simulink model "BimanualCarvingModified"  (R2013a)
settings: Solver=ode4  SolverMode=SingleTasking  StartTime=0.0  StopTime=inf  FixedStep=0.0005  RelTol=1e-3
StartFcn:
  |  warndlg('Dexterit-E models cannot run under simulation. Please compile your model and run it from within Dexterit-E.');set_param(bdroot,'SimulationCommand','stop')
model workspace (MAT data in the model file):
  BKIN_STEP_TIME = 0.0005
  col_x = 1
  col_y = 2
  WIDTH = 3
  HEIGHT = 4
  TARGET_COL = 1
  LOAD = 2
  TRAJ_DURATION_COL = 3
  MAX_LOAD = 2
  FORCE_ON = 1
  HAND_RADIUS = 6
  REST_COL = 4
  TRAINING_COL = 5
  HAND_COLOR = 5
  TARGET_STROKE = 8
  TARGET_RADIUS = 9
  xMaxCursor = 15
  yMaxCursor = 16
  TARGET_COLOR = 7
  START_X = 10
  START_Y = 11
  STIFFNESS_MATERIAL = 3
  MATERIAL_MASS = 4
  MATERIAL_DAMPING = 5
  STIFFNESS_HANDS = 6
  MATERIAL_GOAL_COLOR = 12
  SCALE_VIBRATION = 7
  STONE_WIDTH = 6
  MATERIAL_DUCTILITY = 8
  TARG_COLOR = 1
  TEXT_COLOR = 13
  TEXTBOX_WIDTH = 14
  TEXTBOX_HEIGHT = 15
  ROTATION = 16
  LABEL_TEXT = 17
  LABEL_COLOR = 18
  LABEL_HEIGHT = 19
  ADVANCE_EMG_PLACEMENT = 2
  ADVANCE_EMG_MAX = 3
  EMG_ADVANCE_BUTTON = 1
  EMG_MVC_BUTTON = 2
  START_TRIAL = 3
  END_TRIAL = 4
  MUSC_NUM = 2
  HAND_DISTANCE = 3
  SYN_NUM = 4
  IS_R2_REAL = 5
  R2_SCORE_SD = 6
undefined symbols (not defined in the file or in its folder): slselsubs
libraries: xpclib x9, simulink x6, General x3, KINARM_loads x2, Video x2, KINARM_IO x1, KINARM_EP_loads x1
(part 4 of 6)

== matlab function BimanualCarvingModified/Draw_target/MATLAB Function ==
  data: target input; VCODE output; state_in input; target_type input; opacity_in input; target_display input; x_index input; y_index input; num_states input; stateindices input; target_labels input; KINData input; yWall input; trial_state input; stoneWidth input
function VCODE = fcn(target, state_in, target_type, opacity_in, target_display, x_index, y_index, num_states, stateindices, target_labels, KINData, yWall, trial_state,stoneWidth)

% stateindices should follow this order (depending on target-type):
% 1: fill colour
% 2: stroke colour
% 3: stroke width
% 4: major radius / radius / start point (line)
% 5: minor radius / end point (line)
% 6: orientation angle



% VCODEs are length 70. All units in a VCODE should be SI, e.g. (m) and (rad). Elements in a VCODE are defined as follows:
%
% For all target types:
%  1: target type
%       1 - circle
%       2 - ellipse
%       3 - rectangle
%       4 - line
%       5 - triangle
%       11 - circle with label
%       12 - ellipse with label
%       13 - rectangle with label
%       14 - line with label
%       15 - triangle with label
%  2: target on/off status and target display (which display target will appear on)
%		0 - off
%		1 - on, appearing on both subject and operator displays
%       2 - on, appearing on subject display only
%       3 - on, appearing on operator display only
%  3: x position (m)
%  4: y position (m)
%  5: fill colour (RRGGBB) or texture index
%  6: stroke colour (RRGGBB) or texture index
%  7: stroke width
%  8: reserved for target background ID
%  9: opacity
%
% For circles:
%  10: radius (m)
%
% For ellipses:
%  10: major radius (m)
%  11: minor radius (m)
%  12: orientation of major axis (rad)
%
% For rectangles:
%  10: length (m)
%  11: height (m)
%  12: orientation (rad) (relative to x, y already shown)
%
% For lines:
%  10: endpoint x-axis coordinate relative to start point (m)
%  11: endpoint y-axis coordinate relative to start point (m)
%
% For triangles:
%  10: length (m)
%  11: height (m)
%  12: offset of peak from midpoint of length (m)
%  13: orientation (rad)
%
% For all labelled target types:
%  14: reserved
%  15-64: label characters (indexes in ISO 8859-1 character set)
%  65: label colour (0xRRGGBB), opacity is set by the vcode's opacity (9).
%  66: label height (m)
%  67: reserved
%  68: reserved
%  69: reserved
%  70: reserved

num_targets = 4;
stoneLength = 0.1;

% NOTE: we assume that the STATE and/or OPACITY inputs are vectors. 

% If the length of the input STATE is not the same as the number of targets then make STATE a column vector of the same length as 
% the TARGET input, using the first STATE (i.e. all targets get the same state)
if num_targets == length(state_in)
	state = reshape(state_in, num_targets, 1);
else
	state = state_in(1) * ones(num_targets, 1);
end


% If the length of the input OPACITY is not the same as the number of targets then make OPACITY a column vector of the same length as
% the TARGET input, using the first OPACITY (i.e. all targets get the same opacity)
if num_targets == length(opacity_in)
	opacity = reshape(opacity_in, num_targets, 1);
else
	opacity = opacity_in(1) * ones(num_targets, 1);
end


% Clamping the opacity to [0, 100].
opacity = min(opacity, 100);
opacity = max(opacity, 0);

VCODE = zeros(num_targets, 70);

% Set the target type. Targets with labels have type codes 10 greater than their unlabelled counterparts.
VCODE(:, 1) = target_type + 10;
VCODE(:, 2) = target_display;

VCODE(:, 5) = colourshift(target(1, stateindices(state(1), 1)));
VCODE(:, 6) = colourshift(target(1, stateindices(state(1), 1)));

% Set the opacity value
VCODE(:, 9) = opacity_in(1);
% Target only visible during tracking in trial_state==2
if trial_state==0
    VCODE(:, 5) = colourshift(1000000000);
    VCODE(:, 6) = colourshift(1000000000);
    VCODE(:, 9) = 0;
end


% Stroke width
VCODE(:, 7) = target(1, stateindices(state(1), 3))*0.01 * 2;

VCODE(:, 3) = [-stoneWidth/2;stoneWidth/2;stoneWidth/2;-stoneWidth/2];  % x position (m)
VCODE(:, 4) = [yWall;yWall;yWall+stoneLength;yWall+stoneLength];  % y position (m)

VCODE(:, 10) = [stoneWidth;0;-stoneWidth;0];  % line endpoint in x axis, relative to start (m)
VCODE(:, 11) = [0;stoneLength;0;-stoneLength];  % line endpoint in y axis, relative to start (m)

%{
persistent TargetIndex;
if isempty(TargetIndex), TargetIndex = 1; end
% Set the hand position.
if TargetIndex<=length(xMaterial)
    % Initially draw the whole material from left to right
    % Line beginning
    VCODE(:, 3) = xMaterial(TargetIndex);  % x position (m)
    VCODE(:, 4) = yMaterial(TargetIndex);  % y position (m)
    
    % Line endpoint
    VCODE(:, 10) = xMaterial(TargetIndex+1)-VCODE(:,3);  % line endpoint in x axis, relative to start (m)
    VCODE(:, 11) = yMaterial(TargetIndex+1)-VCODE(:,4);  % line endpoint in y axis, relative to start (m)
else
    % After material is all drawn, update only the changing section
    % Line beginning
    VCODE(:, 3) = xMaterial(MaterialUpdateInd1);  % x position (m)
    VCODE(:, 4) = yMaterial(MaterialUpdateInd1);  % y position (m)
    
    % Line endpoint
    VCODE(:, 10) = xMaterial(MaterialUpdateInd2)-VCODE(:,3);  % line endpoint in x axis, relative to start (m)
    VCODE(:, 11) = yMaterial(MaterialUpdateInd2)-VCODE(:,4);  % line endpoint in y axis, relative to start (m)
end


TargetIndex = min(length(xMaterial)+5,TargetIndex+1);
%}
%{
for ii = 1:num_targets
	% Set the target on/off state. If the state input is 0, the target is off. Users of the VCODE should respect this
	% as an indication that the rest of the VCODE will be uninitialized.
	if (state(ii) <= 0) || (state(ii) > num_states)
		VCODE(ii, 2) = 0;  % target is off
	else
		VCODE(ii, 2) = target_display;  % Default is that target is on; target displays as specified by block mask
	end

	fill_colour_col = stateindices(state(ii), 1);
	stroke_colour_col = stateindices(state(ii), 2);
	stroke_width_col = stateindices(state(ii), 3);
	
	% Set the fill colour. Fill colour currently comes from the GUI in RRRGGGBBB format.
	%{
    if fill_colour_col == 0
		VCODE(ii, 5) = -2^31;
	elseif target(fill_colour_col) < 0
		VCODE(ii, 5) = target(ii, fill_colour_col);
	else
		VCODE(ii, 5) = colourshift(target(ii, fill_colour_col));
    end
    %}
    VCODE(ii,5) = colourshift(1000000000);
	
	% Set the stroke colour. Stroke colour currently comes from the GUI in RRRGGGBBB format.
    if trial_state==1
        if stroke_colour_col == 0
            VCODE(ii, 6) = -2^31;
        elseif target(stroke_colour_col) < 0
            VCODE(ii, 6) = target(ii, stroke_colour_col);
        else
            VCODE(ii, 6) = colourshift( target(ii, stroke_colour_col) );
        end
    else
        % CIRCLE APPEARS ONLY DURING TASK
        VCODE(ii, 6) = colourshift(1000000000);
    end

	% Set the stroke width. if target table index for stroke width is zero, then the stroke width is undefined
	if stroke_width_col == 0
		VCODE(ii, 7) = 0;                   % if stroke width column is 0, then stroke width is 0
	elseif stroke_width_col < 0
		VCODE(ii, 7) = 0.001;               % if stroke width column is -ve, then a 1mm default is chosen
	else
		VCODE(ii, 7) = target(ii, stroke_width_col) * 0.01;  % if stroke width column is +ve, convert width from (cm) in target table to (m)
    end

	% Set the opacity value
	VCODE(ii, 9) = opacity(ii);

	% Set attributes specific to each target type. In the process, note the first state vector column used for label information.
	label_index = 1;

	% Set attributes specific to each target type.
	if target_type == 1

		% Handle circle target:
		radius_col = stateindices(state(ii), 4);
		VCODE(ii, 10)=target(ii, radius_col);  % radius (in m)
	    label_index = 5;

	elseif target_type == 2 || target_type == 3

	    % Handle ellipse or rectangle target:
		major_col = stateindices(state(ii), 4);
		minor_col = stateindices(state(ii), 5);
		orientation_col = stateindices(state(ii), 6);
		
		VCODE(ii, 10) = target(ii, major_col) * 0.01;  % major radius (convert from (cm) in target table to (m))
		VCODE(ii, 11) = target(ii, minor_col) * 0.01;  % minor radius (convert from (cm) in target table to (m))
		if orientation_col == 0
			VCODE(ii, 12) = 0;  % if orientation column is 0, set orientation to 0 rad
		else
			VCODE(ii, 12) = mod(target(ii, orientation_col), 360) * pi / 180.0;  % orientation (convert from (degrees) in target table to (rad))
		end
	    label_index = 7;
	
	elseif target_type == 4

		% Handle line target:
		%xendpoint_col = stateindices(state(ii), 4);
		%yendpoint_col = stateindices(state(ii), 5);
		VCODE(ii, 10) = 0;  % line endpoint in x axis, relative to start (m)
		VCODE(ii, 11) = stateindices(state(ii), 1);  % line endpoint in y axis, relative to start (taken from Target Table)
	    label_index = 6;

	elseif target_type == 5

		% Handle triangle target:
		length_col = stateindices(state(ii), 4);
		height_col = stateindices(state(ii), 5);
		offset_col = stateindices(state(ii), 6);
		orientation_col = stateindices(state(ii), 7);

		VCODE(ii, 10) = target(ii, length_col) * 0.01;  % length (convert from (cm) in target table to (m))

		% If the height column is set to 0 then the triangle is automatically made equilateral, with the base length used as length
		% for all sides. If the height column is non-zero, separate values for height and peak offset are taken from the target table.
		if height_col == 0
			VCODE(ii, 11) = sin(pi / 3.0) * VCODE(ii, 10);  % height for equilateral triangle
			VCODE(ii, 12) = 0;                          % peak offset for equilateral triangle
		else
			VCODE(ii, 11) = target(ii, height_col) * 0.01;  % height (convert from (cm) in target table to (m))
			VCODE(ii, 12) = target(ii, offset_col) * 0.01;  % peak offset (convert from (cm) in target table to (m))
		end

		if orientation_col == 0
			VCODE(ii, 13) = 0;  % if orientation column is 0, set orientation to 0 rad
		else
			VCODE(ii, 13) = mod(target(ii, orientation_col), 360) * pi / 180.0;  % orientation (convert from (degrees) in target table to (rad))
		end
	    label_index = 8;
		
	end
	
	% Copy the label characters to the VCODE.
	for jj = 1:50
		VCODE(ii, jj + 14) = target_labels( target( ii, stateindices(state(ii), label_index) ), jj );
	end

	% Set the label colour. Like other colours, label colour comes from the GUI in RRRGGGBBB format and is converted to a 32-bit
	% 0xRRGGBB value here. If the target column table index for the colour is 0, the label is transparent.
	if stateindices(state(ii), label_index + 1) == 0
		VCODE(ii, 65) = -2^31;
	elseif target( ii, stateindices(state(ii), label_index + 1) ) < 0
		VCODE(ii, 65) = target( ii, stateindices(state(ii), label_index + 1) );
	else
		VCODE(ii, 65) = colourshift( target( ii, stateindices(state(ii), label_index + 1) ) );
	end

	% Set the label height. Label height is converted from (cm) in the target table to (m).
	VCODE(ii, 66) = target( ii, stateindices(state, label_index + 2) ) * 0.01;


	
end
%}
% The colourshift function converts an "RRRGGGBBB" colour value to RRGBB (as an uint32).
function RRGGBBAA = colourshift(RRRGGGBBB)

%this is "no fill"
if RRRGGGBBB == 1000000000
    RRGGBBAA = cast(16777216, 'uint32'); %hex 0x1000000
    return; 
end

blue = cast(mod(RRRGGGBBB, 1000), 'uint32');
green = cast(mod(RRRGGGBBB - blue, 1000000) / 1000, 'uint32');
red = cast((RRRGGGBBB - (green * 1000) - blue) / 1000000, 'uint32');

RRGGBBAA = bitshift(red, 16) + bitshift(green, 8) + blue;

== matlab function BimanualCarvingModified/Trajectory subsystem/Create_Trajectory/Virtual_Trajectory/Extract_Position ==
  settings: fimath=|
      | fimath(...
      | 'RoundMode', 'floor',...
      | 'OverflowMode', 'wrap',...
      | 'ProductMode', 'KeepLSB', 'ProductWordLength', 32,...
      | 'SumMode', 'KeepLSB', 'SumWordLength', 32,...
      | 'CastBeforeSum', false)
  data: u input; position output
function position = fcn(u)

position=[0,0];	%initialization
if length(u)==2	%input is assumed to be (x,y) position, global coordinates, (m)		
	position=u;
else			%input is assumed to be a VCODE
	position(1)=u(3);
	position(2)=u(4);
end

== matlab function BimanualCarvingModified/function ==
  data: KINdata input; trial_state input; MaterialPos output; MaterialTargetPos output; kMaterial input; MaterialMass input; MaterialUpdateInd1 output; MaterialUpdateInd2 output; MaterialDamping input; xStart input; yStart input; xForceRobotL output; yForceRobotL output; HandDistance input; kHands input; xForceRobotR output; yForceRobotR output; yWall output; materialPosY output; ScaleVibration input; stoneWidth input; materialDuctility input; smoothnessScore output; baseScore output
function [MaterialPos,MaterialTargetPos,MaterialUpdateInd1,MaterialUpdateInd2,xForceRobotL,yForceRobotL,xForceRobotR,yForceRobotR,yWall,materialPosY,smoothnessScore,baseScore] = calculate_stuff(KINdata,trial_state,kMaterial,MaterialMass,MaterialDamping,xStart,yStart,HandDistance,kHands,ScaleVibration,stoneWidth,materialDuctility)

dt = 0.0005;

% Ensure material mass and damping are non zero
kMaterial = max(0,kMaterial);
MaterialMass = max(0.001,MaterialMass);
MaterialDamping = max(0,MaterialDamping);

% Position of wall that carves material
yWall = 0.3;
nPoints = 30;
handOffset = 0.02;

% Position of hands
RightHandPos = [KINdata(1,23); KINdata(1,24)];
LeftHandPos = [KINdata(2,23); KINdata(2,24)];
RightHandVel = [KINdata(1,25); KINdata(1,26)];
LeftHandVel = [KINdata(2,25); KINdata(2,26)];
PerpVect = handOffset*[RightHandPos(2)-LeftHandPos(2);RightHandPos(1)-LeftHandPos(1)]/HandDistance;
MiddlePos = mean([LeftHandPos,RightHandPos],2);

% Initial position of material
% MaterialTargetInit = [linspace(-HandDistance/2,HandDistance/2,20); 0.05*sin(linspace(0,pi,20))+0.02];
% MaterialPosUnrotatedInit = [MaterialTargetInit(1,:); MaterialTargetInit(2,:)+ 0.02*sin(linspace(0,10*pi,20))+0.02];

MaterialTargetInit = [linspace(-HandDistance/2,HandDistance/2,nPoints); zeros(1,nPoints)];
MaterialPosUnrotatedLeftInit = [-HandDistance/2*ones(1,5); linspace(-handOffset,0,5)];
MaterialPosUnrotatedTopInit = [MaterialTargetInit(1,:); 0.005*rand(1,nPoints)-0.005/2 + 0.005];
MaterialPosUnrotatedRightInit = [HandDistance/2*ones(1,5); linspace(0,-handOffset,5)];
MaterialPosUnrotatedInit = [MaterialPosUnrotatedLeftInit MaterialPosUnrotatedTopInit MaterialPosUnrotatedRightInit];

% Make sure edges are aligned!
% MaterialPosUnrotatedInit(2,1) = MaterialTargetInit(2,1); MaterialPosUnrotatedInit(2,end) = MaterialTargetInit(2,end);

persistent trial_state_record; persistent TrialTime; persistent yMaterialVel; persistent xMaterialVel; persistent Counter; persistent Counter2; persistent MaterialPosUnrotated; persistent LeftSpringPosRecord; persistent RightSpringPosRecord; persistent baseSmoothnessScore;
if isempty(trial_state_record), trial_state_record=0; TrialTime=0; yMaterialVel=zeros(1,size(MaterialPosUnrotatedInit,2)); xMaterialVel=zeros(1,size(MaterialPosUnrotatedInit,2)); Counter=1; Counter2=0; MaterialPosUnrotated=MaterialPosUnrotatedInit; LeftSpringPosRecord=zeros(2,1); RightSpringPosRecord=zeros(2,1);baseSmoothnessScore = 1;end;

if trial_state~=1
    % Timer is zero besides during task
    TrialTime = 0;
end
if trial_state_record==0 && trial_state==1
    % Reset time after trial begins
    TrialTime = 0;
    
    % Reset material
    baseSmoothnessScore = trapz(MaterialPosUnrotatedInit(1,6:end-5),abs(MaterialPosUnrotatedInit(2,6:end-5)-mean(MaterialPosUnrotatedInit(2,6:end-5))))/nPoints;
    MaterialPosUnrotated = MaterialPosUnrotatedInit;
    yMaterialVel=zeros(1,size(MaterialPosUnrotated,2));
    xMaterialVel=zeros(1,size(MaterialPosUnrotated,2));
    
    % Reset counter
    Counter = 0;
    Counter2 = 0;
end




% Position where hand is connected to other hand
LeftSpringPos = (LeftHandPos-MiddlePos)/norm(LeftHandPos-MiddlePos)*HandDistance/2+MiddlePos;
RightSpringPos = (RightHandPos-MiddlePos)/norm(RightHandPos-MiddlePos)*HandDistance/2+MiddlePos;
% Velocity of spring centres
LeftSpringVel = (LeftSpringPos-LeftSpringPosRecord)/dt;
RightSpringVel = (RightSpringPos-RightSpringPosRecord)/dt;
% Force to couple hands together
LeftForceHands = kHands*(LeftSpringPos-LeftHandPos) + 5*(LeftSpringVel-LeftHandVel);
RightForceHands = kHands*(RightSpringPos-RightHandPos) + 5*(RightSpringVel-RightHandVel);

% Angle between hands
AngleHands = atan2(RightHandPos(2)-LeftHandPos(2),RightHandPos(1)-LeftHandPos(1));

% x-y position of material
MaterialPos = [cos(AngleHands),-sin(AngleHands);sin(AngleHands),cos(AngleHands)]*MaterialPosUnrotated + repmat(MiddlePos+PerpVect,1,size(MaterialPosUnrotatedInit,2));
MaterialTargetPosPre = [cos(AngleHands),-sin(AngleHands);sin(AngleHands),cos(AngleHands)]*MaterialTargetInit + repmat(MiddlePos+PerpVect,1,size(MaterialTargetInit,2));
MaterialTargetPos = MaterialTargetPosPre(:,[1 nPoints]);

% Find all points of contact where material is beyond wall
% Contacts = find(MaterialPos(2,:)>yWall);

% Find all points of contact where material is within grindstone
Contacts = find(MaterialPos(2,:)>yWall & MaterialPos(1,:)>-stoneWidth/2 & MaterialPos(1,:)<stoneWidth/2);

% CALCULATE CONTACTS AND FORCES
LeftForceTotal=zeros(2,1); RightForceTotal=zeros(2,1); 
ForceMaterialY=zeros(1,size(MaterialPos,2));
ForceMaterialX=zeros(1,size(MaterialPos,2));

MaterialUpdateInd1 = 1;
MaterialUpdateInd2 = 2;
for ContactInd=1:size(MaterialPos,2)
    
    % Contact between wall and material
    if ismember(ContactInd,Contacts) %&& ContactInd>1 && ContactInd<size(MaterialPos,2)
        % Position to base of material in contact
        BasePos = MaterialPos(:,ContactInd+1) - MaterialPos(:,ContactInd-1);
        BasePerp = [BasePos(2);BasePos(1)]/norm(BasePos)*materialDuctility;
        
        % Position vector of left and right hands w.r.t. middle
        LeftHandToMid = (LeftHandPos-MiddlePos);
        RightHandToMid = (RightHandPos-MiddlePos);
              
        % Force, torque from wall
        Force = [0; kMaterial*(yWall-MaterialPos(2,ContactInd))];
        Torque = cross([MaterialPos(:,ContactInd)-MiddlePos; 0],[Force; 0]);
        ForceDeform = BasePerp * kMaterial*(yWall-MaterialPos(2,ContactInd));
        % Rotate deformation force onto unrotated coordinates
        ForceDeform = [cos(-AngleHands),-sin(-AngleHands);sin(-AngleHands),cos(-AngleHands)]*ForceDeform;
        ForceMaterialY(ContactInd) = ForceDeform(2);
        ForceMaterialX(ContactInd) = ForceDeform(1);
        
        % Rotational force on both hands
        AngleTorque = atan2(LeftHandToMid(2),LeftHandToMid(1));
        LeftTorque = (Torque(3)/norm(LeftHandToMid))*[cos(AngleTorque),-sin(AngleTorque);sin(AngleTorque),cos(AngleTorque)]*[0; 1];
        RightTorque = (Torque(3)/norm(RightHandToMid))*[cos(AngleTorque),-sin(AngleTorque);sin(AngleTorque),cos(AngleTorque)]*[0; -1];
              
        % Total force on each hand (translation+rotation)
        LeftForceTotal = LeftForceTotal+LeftTorque+Force;
        RightForceTotal = RightForceTotal+RightTorque+Force;
        
        MaterialUpdateInd1 = ContactInd;
        MaterialUpdateInd2 = ContactInd;
    end
    
    % If hand contacts wall, exert force feedback but no material deformation
%     if ismember(ContactInd,Contacts) && (ContactInd==1 || ContactInd==size(MaterialPos,2))
%         % Force, torque from wall
%         Force = [0; kMaterial*(yWall-MaterialPos(2,ContactInd))];
%         % Total force on each hand (translation+rotation)
%         LeftForceTotal = LeftForceTotal+Force;
%         RightForceTotal = RightForceTotal+Force;
%     end
end
    

        %{
        % Force feedback from material
        FxMaterial = kMaterial*(xNearest-xHand)*double(yHand-yNearest>0);
        FyMaterial = kMaterial*(min(0,yNearest - yHand));

        % Deformation of material
        %yMaterial(NearestInd+IndexOffset) = yMaterial(NearestInd+IndexOffset)-DeformScale*(1-abs(x1-xNearest)/abs(x1-x2))*FyMaterial;
        %yMaterial(NearestInd+1+IndexOffset) = yMaterial(NearestInd+1+IndexOffset)-DeformScale*(1-abs(x2-xNearest)/abs(x1-x2))*FyMaterial;
        
        MaterialUpdateInd1 = NearestInd+IndexOffset;
        MaterialUpdateInd2 = NearestInd+1+IndexOffset;
        
        % Force to move material
        %ForceMaterial(MaterialUpdateInd1) = -(1-abs(x1-xNearest)/abs(x1-x2))*FyMaterial;
        %ForceMaterial(MaterialUpdateInd2) = -(1-abs(x2-xNearest)/abs(x1-x2))*FyMaterial;
        ForceMaterial(MaterialUpdateInd1) = -(1-abs(x1-xHand)/abs(x1-x2))*FyMaterial;
        ForceMaterial(MaterialUpdateInd2) = -(1-abs(x2-xHand)/abs(x1-x2))*FyMaterial;
        
        yMaterialPosition = ((y2-y1)/(x2-x1))*(xHand-x1)+y1;
        %}

if Counter<size(MaterialPos,2)  
    MaterialUpdateInd1 = Counter;
    MaterialUpdateInd2 = Counter+1;
end

VibrationForceLeft=zeros(2,1);
VibrationForceRight=zeros(2,1);
if norm(LeftForceTotal)+norm(LeftForceTotal)>0
    VibrationForceLeft = [0; ScaleVibration*(norm(LeftForceTotal)+norm(LeftForceTotal))*sin(2*pi*15*TrialTime)];
    VibrationForceRight = [0; ScaleVibration*(norm(RightForceTotal)+norm(RightForceTotal))*sin(2*pi*15*TrialTime)];
end

% Force to send as feedback
xForceRobotL = LeftForceHands(1)+LeftForceTotal(1)+VibrationForceLeft(1);
yForceRobotL = LeftForceHands(2)+LeftForceTotal(2)+VibrationForceLeft(2);
xForceRobotR = RightForceHands(1)+RightForceTotal(1)+VibrationForceRight(1);
yForceRobotR = RightForceHands(2)+RightForceTotal(2)+VibrationForceRight(2);


% Visually update and record material
% yMaterialUpdate1 = 0;%yMaterial(max(1,min(length(xMaterialInit),MaterialUpdateInd1)));
% yMaterialUpdate2 = 0;%yMaterial(max(1,min(length(xMaterialInit),MaterialUpdateInd2)));

% materialPosX = MaterialPosUnrotated(1,6:2:end-5);
materialPosY = MaterialPosUnrotated(2,6:end-5);
smoothnessScore = trapz(MaterialPosUnrotated(1,6:end-5),abs(MaterialPosUnrotated(2,6:end-5)-mean(MaterialPosUnrotated(2,6:end-5))))/nPoints;
baseScore = baseSmoothnessScore;

% Material dynamics
MaterialPosUnrotated(1,:) = MaterialPosUnrotated(1,:) + xMaterialVel*dt;
xMaterialVel = (1-MaterialDamping*dt/MaterialMass)*xMaterialVel + (dt/MaterialMass)*ForceMaterialX;
MaterialPosUnrotated(2,:) = MaterialPosUnrotated(2,:) + yMaterialVel*dt;
yMaterialVel = (1-MaterialDamping*dt/MaterialMass)*yMaterialVel + (dt/MaterialMass)*ForceMaterialY;
     
% Record positions of spring centers
LeftSpringPosRecord = LeftSpringPos;
RightSpringPosRecord = RightSpringPos;

% Record variable
trial_state_record = trial_state;
Counter2 = Counter2+1;
if mod(Counter2,2)==0
    Counter = Counter+1;
end

TrialTime = TrialTime+dt;

== matlab function BimanualCarvingModified/Trajectory subsystem/Create_Trajectory/Virtual_Trajectory/Extract_Position1 ==
  settings: fimath=|
      | fimath(...
      | 'RoundMode', 'floor',...
      | 'OverflowMode', 'wrap',...
      | 'ProductMode', 'KeepLSB', 'ProductWordLength', 32,...
      | 'SumMode', 'KeepLSB', 'SumWordLength', 32,...
      | 'CastBeforeSum', false)
  data: u input; position output
function position = fcn(u)

position=[0,0];	%initialization
if length(u)==2	%input is assumed to be (x,y) position, global coordinates, (m)		
	position=u;
else			%input is assumed to be a VCODE
	position(1)=u(3);
	position(2)=u(4);
end

== matlab function BimanualCarvingModified/Trajectory subsystem/calculate robot scaling/MATLAB Function ==
  data: robot_type input; scaling output; exo_scaling input; ep_scaling input
function scaling = fcn(robot_type, exo_scaling, ep_scaling)
%#codegen

scaling = [0, 0];

%0 = EXO, 1 = EP, 2 = NHP
for n=1:2
    if robot_type(n) == 1
        scaling(n) = ep_scaling(n);
    else
        scaling(n) = exo_scaling(n);
    end
end

== stateflow chart BimanualCarvingModified/Trajectory subsystem/Create_Trajectory/Virtual_Trajectory/VirtualTrajectory ==
  state Initialization/
    virt_pos = reset_pos;
    // this initialization ensures that the virtual position
    // starts off as something reasonable
    traj_status = 0;   // initialize trajectory status
  state main/
    state wait_for_trigger/
      reset_controller = 0;
    state wait_1_ms_b/
      // wait for controller
      // to be reset
    state on_ramp/
      entry: tick = 0;    // initialize the tick counter
      reset_controller = 0;
      final_pos = target_pos;   // set the final position of the trajectory
      start_pos = virt_pos;   // set the start position of the trajectory
      duration = input_duration;   // store the duration of the trajectory
      traj_status = 1;   // indicate an ongoing trajectory
      during:
      on e_clk: tick++;
      // the trajectory velocity will have a bell shaped profile
      trajectory_shape = tick/duration-sin(2*pi*tick/duration)/(2*pi);
      virt_pos[1] = start_pos[1] + (final_pos[1] - start_pos[1]) * trajectory_shape;
      virt_pos[2] = start_pos[2] + (final_pos[2] - start_pos[2]) * trajectory_shape;
    main -> wait_1_ms_b [order 1] : [(robot_enabled == 1) && (traj_status == -1)]/
        | traj_status = 1;
        | virt_pos = reset_pos;
        | reset_controller = 1;
        | // trajectory was halted and
        | //is now being re-started
    wait_for_trigger -> (junction 20) : e_start
    (junction 20) -> wait_for_trigger [order 2]
    wait_1_ms_b -> (junction 20) : after(1, e_clk)
    (junction 20) -> on_ramp [order 1] : [input_duration>0]
    on_ramp -> wait_for_trigger [order 2] : [robot_enabled == 0]/
        | traj_status = -1;
        | // robot disabled
    on_ramp -> wait_for_trigger [order 1] : after(duration, e_clk)/
        | traj_status = 0
        | // trajectory completed
  state wait_1_ms/
    // wait for controller
    // to be reset
  state task_not_running/
    // wait for task_status to change
    // keep updating virt_pos so that the feedback
    // controller output, which is filtered, does not become
    // huge, resulting in a 'bump' if we don't do this.
    traj_status = 0;
    reset_controller = 0;
    during:
    virt_pos = reset_pos;
  (default) -> Initialization
  Initialization -> wait_for_trigger
  wait_1_ms -> wait_for_trigger : after(1, e_clk)
  task_not_running -> wait_1_ms : [task_status > 0]/
      | reset_controller = 1;
      | // task is running again,
      | // so reset position controller
  main -> task_not_running [order 1] : [task_status == 0]/
      | // means that run_status == 0
      | // AND that torque scaling at
      | // end of task is finished
  data: input_duration input double; target_pos input double size=[1 2]; tick local double; duration local double; reset_pos input double size=[1 2]; task_status input double; pi constant double =3.14159265358979; trajectory_shape local double; virt_pos output double size=[1 2]; traj_status output double; robot_enabled input double; start_pos local double size=[1 2]; final_pos local double size=[1 2]; reset_controller output double
  events: e_clk input RISING_EDGE_EVENT; e_start input RISING_EDGE_EVENT

== matlab function BimanualCarvingModified/Trajectory subsystem/Create_Trajectory/get_arm_info ==
  settings: fimath=|
      | fimath(...
      | 'RoundMode', 'floor',...
      | 'OverflowMode', 'wrap',...
      | 'ProductMode', 'KeepLSB', 'ProductWordLength', 32,...
      | 'SumMode', 'KeepLSB', 'SumWordLength', 32,...
      | 'CastBeforeSum', false)
  data: position output; task_status output; use_dom_hand input; kinarm_data input; run_status input; scaling input; robot_enabled output
function [position, task_status, robot_enabled]  = fcn(use_dom_hand, kinarm_data, run_status, scaling)
%
% get current hand position and robot enabled status
%
% May 2009
%

hpx_index = 23;
hpy_index = 24;
robot_disabled_index = 37;

%determine which arm to apply the load to
dominant_hand=kinarm_data(3,1);						%kinarm_data(3,1) tells which arm is the dominant arm
if use_dom_hand == 1
	feedback_arm = dominant_hand;
else
	feedback_arm = 3 - dominant_hand;
end

hpx = kinarm_data( feedback_arm, hpx_index );
hpy = kinarm_data( feedback_arm, hpy_index );
position = [hpx hpy];

if kinarm_data( feedback_arm, robot_disabled_index ) == 0;
    robot_enabled = 1;
else
    robot_enabled = 0;
end

% if the task has stopped/paused (i.e. run_status == 0) AND the torques outputs
% have scaled down to 0, then set the task_status = 0.
if run_status == 0 && scaling(feedback_arm) == 0
    task_status = 0;
else
    task_status = 1;
end

== matlab function BimanualCarvingModified/Trajectory subsystem/KINARM_EP_Position_Controller/FF_FB_Position_Controller ==
  settings: fimath=|
      | fimath(...
      | 'RoundMode', 'floor',...
      | 'OverflowMode', 'wrap',...
      | 'ProductMode', 'KeepLSB', 'ProductWordLength', 32,...
      | 'SumMode', 'KeepLSB', 'SumWordLength', 32,...
      | 'CastBeforeSum', false)
  data: Force_FB output; use_dom_hand input; kinarm_data input; setpoint_angles input; setpoint_vel input; setpoint_acc input; Force_FF output; Secondary_Encoders_Used input; inertia_option_for_FF input; primary_encoder_data input; gain_choice input; ForceOn input; xForceRobotL input; yForceRobotL input; xForceRobotR input; yForceRobotR input
function [Force_FB, Force_FF] = fcn(use_dom_hand, kinarm_data, setpoint_angles, setpoint_vel, setpoint_acc, Secondary_Encoders_Used, inertia_option_for_FF, primary_encoder_data, gain_choice, ForceOn,xForceRobotL,yForceRobotL,xForceRobotR,yForceRobotR)
% This block supports the Embedded MATLAB subset.
% See the help menu for details. 
% set point is joint angles in global coordinates

% inertia_option_for_FF sets the options for which inertias to include for 
% the feed-forward model
%	0 - none
%	1 - KINARM robot only

% gain_choice sets the options for which proportional gains to use for the
% controller (does not affect the gains when secondary encoders are used)
%	1 - Standard Movement  == Highest stiffness. For primary encoders only, this is quite underdamped.
%	2 - Step Response == Reduced overshoot for primary encoders only, and lower stiffness.  Same as above for secondary encoders.

%{
L1_index = 1;				% L1 (m)
L2_index = 2;				% L2(m)
ORIENT_index = 6;			% 1=right	2=left
L1Ang_index = 17;			% L1 angle
L2Ang_index = 18;			% L2 Angle
L1Vel_index = 19;			% L1 angle
L2Vel_index = 20;			% L2 Angle

Force_FF = [0 0 0 0];
Force_FB = [0 0 0 0];
%}

%determine which arm to apply the load to
dominant_hand=kinarm_data(3,1);						%kinarm_data(3,1) tells which arm is the dominant arm
if use_dom_hand==1
	arm=dominant_hand;
else
	arm=3-dominant_hand;
end

%{

L1 = kinarm_data( arm, L1_index );
L2 = kinarm_data( arm, L2_index );
L1Ang = kinarm_data( arm, L1Ang_index );
L2Ang = kinarm_data( arm, L2Ang_index );
L1Vel = kinarm_data( arm, L1Vel_index );
L2Vel = kinarm_data( arm, L2Vel_index );
theta=[L1Ang; L2Ang];
thetavel=[L1Vel; L2Vel];
theta_primary = primary_encoder_data(arm, 1:2)';
thetavel_primary = primary_encoder_data(arm, 3:4)';

% Proportional Gain
if gain_choice == 1         %If the "standard movement" gain choice is selected:
    Kp = [200 0; 0 200];	%proportional gain for KINARM EP robot, primary encoders only - high stiffness
else
    Kp = [85 0; 0 85];		%proportional gain for KINARM EP robot, primary encoders only - reduced overshoot
end
Kp_1 = [0 0; 0 0];			%proportional gain for KINARM EP robot, primary encoders if used in conjunction with secondary
Kp_2 = [1 0; 0 1];		%proportional gain for KINARM EP robot, secondary encoders if used in conjunction with primary

% Derivative gain
Kv = [3.5 0; 0 3.5];		% Derivative gain for KINARM EP robot, primary encoders only				
Kv_1 = [2.5 0; 0 2.5];		% Derivative gain for KINARM EP robot, primary encoders if used in conjunction with secondary
Kv_2 = [6 0; 0 6];          % Derivative gain for KINARM EP robot, secondary encoders if used in conjunction with primary	



error = setpoint_angles - theta;
error_vel = setpoint_vel - thetavel;

error_primary = setpoint_angles - theta_primary;
error_vel_primary = setpoint_vel - thetavel_primary;

% THE FOLLOWING ARE TYPICAL VALUES FOR THE KINARM End Point robot (Rev1)
I1_prox		= 0.018;			%inertia of KINARM segment 1, kg-m^2 at shoulder
I2_5_prox	= 0.034;			%inertia of KINARM segments 2&5, kg-m^2 at elbow
I3_prox		= 0.014;			%inertia of KINARM segment 3, kg-m^2 at elbow
I4_prox		= 0.022;			%inertia of KINARM segment 4, kg-m^2 at shoulder
Im1 = 0.0047;			%inertia of motor 1, after 6x gear ratio, kg-m^2
Im2 = 0.0047;			%inertia of motor 2, after 6x gear ratio, kg-m^2
M2 = 0.62;				%mass of KINARM segment2 and 5 (kg)
M4 = 0.80;				%mass of segment 4 (kg)
L3 = 0.187;				%crank length (m)
delta = 0;				%0 degrees, angle between segments 2 and 5
x2 = 0.20;				%center of mass of segments 2+5 (m)
x4 = 0.12;				%center of mass of segment 4 (m)



theta2_1 = setpoint_angles(2) - setpoint_angles(1);
sin21 = sin(theta2_1);
cos21 = cos(theta2_1);
sin51 = sin(theta2_1 - delta);
cos51 = cos(theta2_1 - delta);

% The following equations implement the equations of motion for the KINARM robot
% For simplicity, we have ignored the off-axis components of inertia due to their
% negligible contributions
A = I1_prox + I4_prox + Im1 + M2*L1^2;
B = M2*L1*(x2*cos21) + M4*L3*(x4*cos51);
D = I2_5_prox + I3_prox + Im2 + M4*L3^2;
C = M2*L1*(x2*sin21) + M4*L3*(x4*sin51);

M = [A B; B D];	%inertial matrix
CC = [0 -C; C 0] * diag(setpoint_vel);	%coriolis and centripetal forces

if inertia_option_for_FF == 0;			%no feed-forward control
	TRQ_FF = [0; 0];
else
	TRQ_FF = M*setpoint_acc + CC*setpoint_vel;
end

if Secondary_Encoders_Used(arm) == 0
	% Only use primary encoder feedback
	TRQ_FB = Kp*error + Kv*error_vel;
else
	% Use both primary and secondary encoders - note: secondary encoder information under these conditions is contained error and error_vel
	TRQ_FB = Kp_2*error + Kv_2*error_vel + Kp_1*error_primary + Kv_1*error_vel_primary;
end

%convert torques (applied to links) to forces (applied at end-point);
A1 = -L1*sin(L1Ang);
A2 = L1*cos(L1Ang);
A3 = -L2*sin(L2Ang);
A4 = L2*cos(L2Ang);

F_FF = [A1 A2; A3 A4] \ TRQ_FF;
F_FB = [A1 A2; A3 A4] \ TRQ_FB;
%}

%%%%%%%%%%%%%%%%%%%%%%%%%%%%%%%%%%%%%%%%%%%%%%%%%%%%%%%%%%%%%%%%%%%%%%%%%%%
xPos = kinarm_data(arm,23);
yPos = kinarm_data(arm,24);
xVel = kinarm_data(arm,25);
yVel = kinarm_data(arm,26);



% FINAL FORCE CHECK
if ForceOn==1
    % Send force
    F_FBL = [xForceRobotL; yForceRobotL]; % SET WHEN EVERYTHING IS OKAY
    F_FBR = [xForceRobotR; yForceRobotR]; % SET WHEN EVERYTHING IS OKAY
    %F_FB = [0; 0]; % do not send force yet
else
    % No force
    F_FBL = [0; 0];
    F_FBR = [0; 0];
end
F_FF = [0; 0];

%%%%%%%%%%%%%%%%%%%%%%%%%%%%%%%%%%%%%%%%%%%%%%%%%%%%%%%%%%%%%%%%%%%%%%%%%%%


% Flatten any bad values to 0.
if F_FF(1) ~= F_FF(1)
    F_FF(1) = 0;
end

if F_FF(2) ~= F_FF(2)
    F_FF(2) = 0;
end

if F_FBL(1) ~= F_FBL(1)
    F_FBL(1) = 0;
end

if F_FBL(2) ~= F_FBL(2)
    F_FBL(2) = 0;
end

if F_FBR(1) ~= F_FBR(1)
    F_FBR(1) = 0;
end

if F_FBR(2) ~= F_FBR(2)
    F_FBR(2) = 0;
end

%apply the forces to the correct arm 
Force_FF = [F_FF' 0 0];
Force_FB = [F_FBR' F_FBL'];

== matlab function BimanualCarvingModified/Trajectory subsystem/KINARM_EP_Position_Controller/Get_kinematics_EP/xy_to_segment_angles_EP ==
  settings: fimath=|
      | fimath(...
      | 'RoundMode', 'floor',...
      | 'OverflowMode', 'wrap',...
      | 'ProductMode', 'KeepLSB', 'ProductWordLength', 32,...
      | 'SumMode', 'KeepLSB', 'SumWordLength', 32,...
      | 'CastBeforeSum', false)
  data: use_dom_hand input; kinarm_data input; u input; SEGMENT_ANG output; robot_calib input
function SEGMENT_ANG  = fcn(use_dom_hand, kinarm_data, u, robot_calib)

% This function converts an endpoint finger-tip position or local joint angle (shoulder, elbow) 
% to (L1Ang, L2Ang) angles for a KINARM robot where L1Ang and L2Ang are the global angles of L1 and L2  
% Note: these equations were taken from a source which defined theta1 as the global angle of L1 (i.e. theta1 = L1Ang
% and L2_L1Ang = local angle of L2 WRT L1 (but always in a R.H. coordinate frame).  So L2_L1Ang = L2Ang - L1Ang.
% Also note that we need to correct for L2_ptr

% angles_or_XY sets the options for which coordinate system to use
%	1 - (x, y) coordinates
%	2 - local coordinate joint angles (shoulder, elbow)

% NEED TO GET SHOULDER AND ELBOW ANGLE OFFSETS FROM CALIBRATION WHEN THESE BECOME AVAILABLE.
% For the KINARM End-Point robot I have assumed certain values, which will hold unless the robot
% is mounted at an angle relative to global.
% Need to decide how to deal with this for the Exoskeleton lab.

L1_index = 1;				% L1 (m)
L2_index = 2;				% L2(m)
L2ptr_index = 3;			% L2ptr(m)
SHO_ORIGIN_X_index = 4;		% shoulder origin, x position
SHO_ORIGIN_Y_index = 5;		% shoulder origin, y position
ORIENT_index = 6;			% 1=right	2=left


%determine which arm to apply the load to
dominant_hand=kinarm_data(3,1);						%kinarm_data(3,1) tells which arm is the dominant arm
if use_dom_hand==1
	arm=dominant_hand;
else
	arm=3-dominant_hand;
end

ORIENTATION = kinarm_data( arm, ORIENT_index);

% To be consistent with the Exoskeleton, the shoulder and elbow angles are stored in a 
% 'local' coordinate frame from the robot's perspective.  The right End-Point robot is 
% constructed the same a left KINARM Exoskeleton and vice-versa.  So the 'local' coordinate
% frame for a R.H. KINARM EP robot is actually a left-handed coordinate frame.
Sho_offset = robot_calib(1, arm);		% value stored in calibration in a 'local' coordinate frame.

position=[0,0];	%initialization
if length(u)==2	%input is assumed to be (x,y) position, global coordinates, (m)
    if size(u,1) == 1;
        position=u;
    else
        position=u';
    end
else			%input is assumed to be a VCODE
    position(1)=u(3);
    position(2)=u(4);
end


% calculate theta from (x,y)
L1 = kinarm_data( arm, L1_index );
L2 = kinarm_data( arm, L2_index );
L2ptr = kinarm_data( arm, L2ptr_index );
SHO_ORIGIN_X = kinarm_data( arm, SHO_ORIGIN_X_index );
SHO_ORIGIN_Y = kinarm_data( arm, SHO_ORIGIN_Y_index );

x = position(1) - SHO_ORIGIN_X;
y = position(2) - SHO_ORIGIN_Y;

L2_temp = sqrt(L2^2 + L2ptr^2);
L2_ptr_angle_shift = atan2(L2ptr, L2);			%

% The following calculation assumes that the (local) elbow angle is 
% never less than 0 (i.e. L2_L1Ang > 0 for right-handed Exoskeleton, or LEFT-HANDED End-Point, and 
% L2_L1Ang < 0 for  left-handed Exoskelton or RIGHT-HANDED End-Point).  These are always true if L2ptr > 0.  
% If L2ptr < 0, then two solutions exist, however, the one with (local) 
% elbow_angle > 0 is chosen.  
% In addition, temp is limited to +-1 to avoid an error using acos.  
% Originally this was simple clipping, but the infinite slope at acos(1)
% created instability problems, so tanh(temp + temp^3/3...) was added to 
% smooth out the transition.  The difference in angle is < 1 degree with 
% elbow angle > 30 degrees.  As the elbow extends further, the 'error' 
% is <20 degrees when full extension should theoretically happen.  For 
% L1 = 0.3m and L2 = 0.4m, the end-point error with an input point
% that in theory requires full extension is <1cm.  This end-point error
% is < 1mm when the desired endpoint is >66cm out.
% Note: tanh(temp + temp^3/3...) provides a sharper transition than 
% tanh(temp), which in turn provides a shaper one than atan(temp)
% The more terms in the tanh(temp...) series, the greater the cutoff
temp = (x^2 + y^2 - L1^2 - L2_temp^2) / (2*L1*L2_temp);
% 	temp = sign(temp) * min(abs(temp), 1);          %Not used to avoid infinite slope issue for subsequent acos
temp = tanh(temp + temp^3/3 + temp^5/5 + temp^7/7 + temp^9/9 + temp^11/11);
L2_L1Ang = acos( temp );

% if ORIENTATION == 2 %left-handed KINARM Exoskeleton 
if ORIENTATION == 1 %right-handed KINARM End-Point robot
    L2_L1Ang = -L2_L1Ang;
    L2_ptr_angle_shift = -L2_ptr_angle_shift;
end
sint = sin(L2_L1Ang);
cost = cos(L2_L1Ang);
L1Ang = atan2( ( -x*L2_temp*sint + y *(L1 + L2_temp*cost) ) , ( y*L2_temp*sint + x *(L1 + L2_temp*cost) ) );

% Likewise, there are multiple solutions for the inverse kinematics for 
% L1Ang as well. We know (based on possible arm configurations) which is 
% the correct solution for right-handed versus left-handed KINARMs.
% Sho_offset is in local coordinates.  It is translated to global as  
% L1_offset.  For "left" robots (i.e. left Exo and right EP), 
% L1Ang = -ShoAng + pi.  
% For the KINARM End-Point robot, working from the calibration 
% position (i.e. when L1Ang = L1_Offset), we know that the L1 link cannot 
% point directly backwards into the K-box.  Which for the left KINARM EP is 
% a rotation of -3/4pi or +5/4pi and for the right it is -5/4pi or +3/4pi.

if ORIENTATION == 2 
	% left-handed KINARM End_point
    L1_offset = Sho_offset;
    if L1Ang < (L1_offset - 3/4*pi) 
        L1Ang = L1Ang + 2*pi;
    elseif L1Ang > (L1_offset + 5/4*pi)
        L1Ang = L1Ang - 2*pi;
    end
else
    L1_offset = -Sho_offset + pi;
    if L1Ang < (L1_offset - 5/4*pi) 
        L1Ang = L1Ang + 2*pi;
    elseif L1Ang > (L1_offset + 3/4*pi)
        L1Ang = L1Ang - 2*pi;
    end

end

L2Ang = L1Ang + L2_L1Ang - L2_ptr_angle_shift;

SEGMENT_ANG = [L1Ang; L2Ang];
